simulink model "respuesta_al_escalon"  (R2021a)
settings: Solver=VariableStepAuto  StartTime=0.0  StopTime=50  RelTol=1e-3
libraries: instrumentseriallib x2
settings Model: Creator=Claudio  LastModifiedBy=ASUS
settings DebuggingCC: UnderspecifiedInitializationDetection=Classic  MergeDetectMultiDrivingBlocksExec=none
settings ModelReferenceCC: PropagateSignalLabelsOutOfModel=off

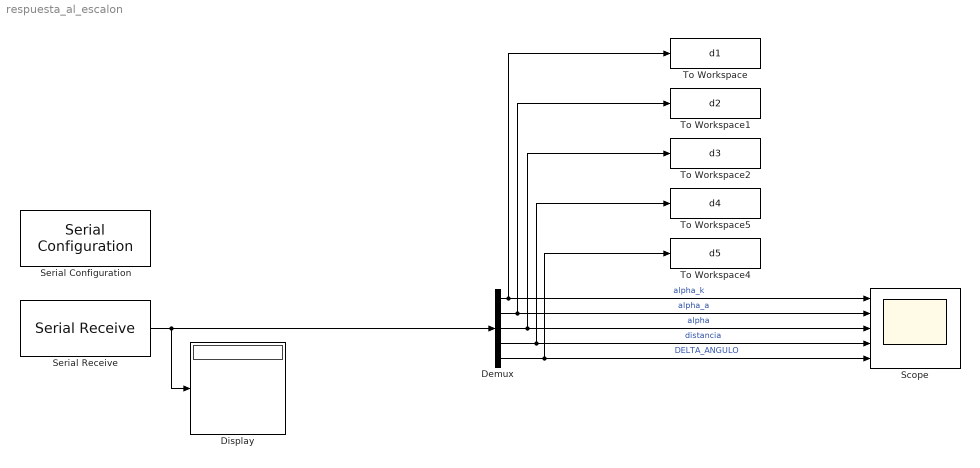
== system respuesta_al_escalon ==
  Demux : Demux  Outputs=5
  Display : Display
  Scope : Scope  NumInputPorts=5
  Serial Configuration : instrumentseriallib/Serial Configuration  Priority=-200000  Port=COM3  ComPort=COM3  BaudRate=115200  DataBits=8  Parity=none  StopBits=1  ByteOrder=little-endian  FlowControl=none  Timeout=10  SimulateUsing=Interpreted execution  BlockInModel=on
  Serial Receive : instrumentseriallib/Serial Receive  Priority=1  Port=COM3  ComPort=COM3  DataType=single  SaveDataType=uint8  ToggleHeader=on  Header="[ 97   98   99  100 ]"  ToggleTerminator=off  Terminator=<none>  CustomTerminator=[]  ToggleDataSize=on  DataSize=[5 1]  EnableBlockingMode=on  ActionDataUnavailable=Output last received value  ActionWhenDataUnavailable=Output last received value  CustomValue=0  SampleTime=0.02  SimulateUsing=Interpreted execution  BlockInModel=on
  To Workspace : ToWorkspace  VariableName=d1  SampleTime=-1
      settings: Save2DSignal=2-D array (concatenate along first dimension)
  To Workspace1 : ToWorkspace  VariableName=d2  SampleTime=-1
      settings: Save2DSignal=2-D array (concatenate along first dimension)
  To Workspace2 : ToWorkspace  VariableName=d3  SampleTime=-1
      settings: Save2DSignal=2-D array (concatenate along first dimension)
  To Workspace4 : ToWorkspace  VariableName=d5  SampleTime=-1
      settings: Save2DSignal=2-D array (concatenate along first dimension)
  To Workspace5 : ToWorkspace  VariableName=d4  SampleTime=-1
      settings: Save2DSignal=2-D array (concatenate along first dimension)
  wires:
  Demux/2 -> To Workspace1/1, Scope/2  "alpha_a"
  Demux/1 -> To Workspace/1, Scope/1  "alpha_k"
  Demux/3 -> To Workspace2/1, Scope/3  "alpha"
  Serial Receive/1 -> Demux/1, Display/1
  Demux/5 -> Scope/5, To Workspace4/1  "DELTA_ANGULO"
  Demux/4 -> To Workspace5/1, Scope/4  "distancia"
